simulink model "flightControlSystem"  (R2026b)
settings: Solver=ode3  StopTime=TFinal
PreLoadFcn:
  | InitVars;
undefined symbols (not defined in the file): control_power, feedforward_gains, integrator_limits, MC_PITCH_P, MC_PITCHRATE_D, MC_PITCHRATE_I, MC_PITCHRATE_MAX, MC_PITCHRATE_P, MC_ROLL_P, MC_ROLLRATE_D, MC_ROLLRATE_I, MC_ROLLRATE_MAX, MC_ROLLRATE_P, MC_YAW_P, MC_YAW_TQ_CUTOFF, MC_YAW_WEIGHT, MC_YAWRATE_D, MC_YAWRATE_I, MC_YAWRATE_MAX, MC_YAWRATE_P, MPC_ACC_DECOUPLE, MPC_LAND_ALT1, MPC_LAND_ALT2, MPC_LAND_ALT3, MPC_LAND_CRWL, MPC_LAND_SPEED, MPC_THR_HOVER, MPC_THR_MAX, MPC_THR_MIN, MPC_THR_XY_MARG, MPC_TILTMAX_AIR, MPC_VELD_LP, MPC_XY_P, MPC_XY_VEL_D_ACC, MPC_XY_VEL_I_ACC, MPC_XY_VEL_MAX, MPC_XY_VEL_P_ACC, MPC_Z_P, MPC_Z_VEL_D_ACC, MPC_Z_VEL_I_ACC, MPC_Z_VEL_MAX_DN, MPC_Z_VEL_MAX_UP, MPC_Z_VEL_P_ACC, SampleTime, timestamp
libraries: px4uORBlib x9, vrlib x8, aerolibutil x8, simulink x4, px4Utilslib x4, sharedutil x3, matrix_library x3, raspberrypiutilitieslib x2, px4Peripheralslib x2, sharedtransform x1, px4Sensorslib x1
(part 3 of 4)

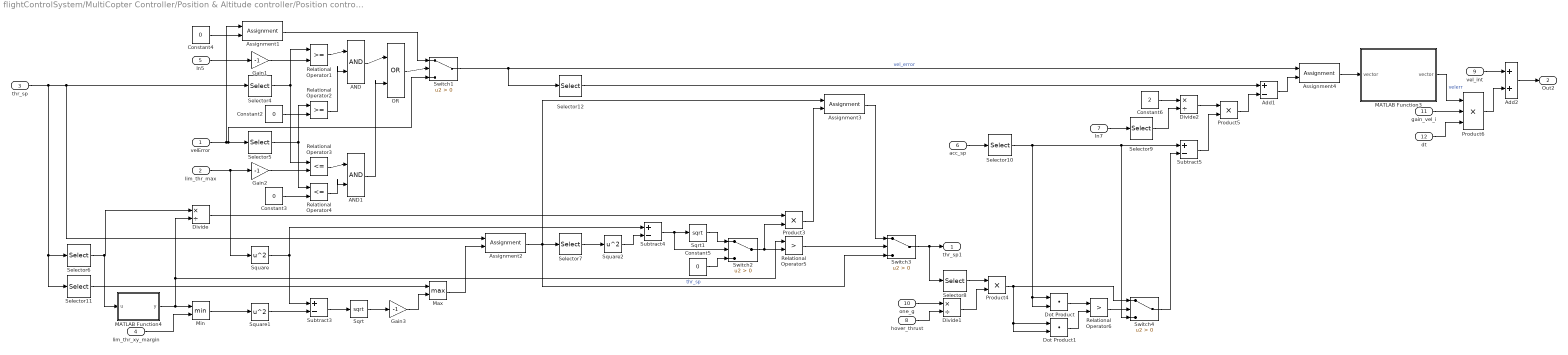
== system flightControlSystem/MultiCopter Controller/Position & Altitude controller/Position controller/Pos/thrust_allocation ==
  velError : Inport
  lim_thr_max : Inport  Port=2
  thr_sp : Inport  Port=3
  lim_thr_xy_margin : Inport  Port=4
  In5 : Inport  Port=5
  acc_sp : Inport  Port=6
  In7 : Inport  Port=7
  hover_thrust : Inport  Port=8
  vel_int : Inport  Port=9
  one_g : Inport  Port=10
  gain_vel_i : Inport  Port=11
  dt : Inport  Port=12
  AND : Logic  IconShape=distinctive  AllPortsSameDT=off  OutDataTypeStr=boolean
  AND1 : Logic  IconShape=distinctive  AllPortsSameDT=off  OutDataTypeStr=boolean
  Add1 : Sum  Inputs=+-
  Add2 : Sum
  Assignment1 : Assignment  DiagnosticForDimensions=Warning  IndexOptions=Index vector (dialog)  Indices=3  OutputSizes=1  RuntimeRangeChecks=off
  Assignment2 : Assignment  DiagnosticForDimensions=Warning  IndexOptions=Index vector (dialog)  Indices=3  OutputSizes=1  RuntimeRangeChecks=off
  Assignment3 : Assignment  DiagnosticForDimensions=Warning  IndexOptions=Index vector (dialog)  Indices=[1,2]  OutputSizes=1  RuntimeRangeChecks=off
  Assignment4 : Assignment  DiagnosticForDimensions=Warning  IndexOptions=Index vector (dialog)  Indices=[1 2]  OutputSizes=1  RuntimeRangeChecks=off
  Constant{2..5} (4 alike) : Constant  Value=0  SampleTime=-1
  Constant6 : Constant  Value=2  SampleTime=-1
  Divide : Product  Inputs=*/
  Divide1 : Product  Inputs=*/
  Divide2 : Product  Inputs=*/
  Dot Product : DotProduct  OutDataTypeStr=Inherit: Inherit via internal rule
  Dot Product1 : DotProduct  OutDataTypeStr=Inherit: Inherit via internal rule
  Gain1 : Gain  Gain=-1
  Gain2 : Gain  Gain=-1
  Gain3 : Gain  Gain=-1
  MATLAB Function3 : MATLAB Function  TreatAsAtomicUnit=on
  MATLAB Function4 : MATLAB Function  TreatAsAtomicUnit=on
  Max : MinMax  Function=max  Inputs=2
  Min : MinMax  Inputs=2
  OR : Logic  Operator=OR  IconShape=distinctive  AllPortsSameDT=off  OutDataTypeStr=boolean
  Product3 : Product
  Product4 : Product
  Product5 : Product
  Product6 : Product  Inputs=3
  Relational Operator1 : RelationalOperator  OutDataTypeStr=boolean  RndMeth=Simplest  InputSameDT=off
  Relational Operator2 : RelationalOperator  OutDataTypeStr=boolean  RndMeth=Simplest  InputSameDT=off
  Relational Operator3 : RelationalOperator  Operator=<=  OutDataTypeStr=boolean  RndMeth=Simplest  InputSameDT=off
  Relational Operator4 : RelationalOperator  Operator=<=  OutDataTypeStr=boolean  RndMeth=Simplest  InputSameDT=off
  Relational Operator5 : RelationalOperator  Operator=>  OutDataTypeStr=boolean  RndMeth=Simplest  InputSameDT=off
  Relational Operator6 : RelationalOperator  Operator=>  OutDataTypeStr=boolean  RndMeth=Simplest  InputSameDT=off
  Selector{6,8,10,12} (4 alike) : Selector  InputPortWidth=3  IndexOptions=Index vector (dialog)  Indices=[1 2]  OutputSizes=1  RuntimeRangeChecks=off
  Selector{4..5,7,11} (4 alike) : Selector  InputPortWidth=3  IndexOptions=Index vector (dialog)  Indices=3  OutputSizes=1  RuntimeRangeChecks=off
  Selector9 : Selector  InputPortWidth=3  IndexOptions=Index vector (dialog)  Indices=1  OutputSizes=1  RuntimeRangeChecks=off
  Sqrt : Sqrt
  Sqrt1 : Sqrt
  Square : Math  Operator=square
  Square1 : Math  Operator=square
  Square2 : Math  Operator=square
  Subtract3 : Sum  Inputs=+-
  Subtract4 : Sum  Inputs=+-
  Subtract5 : Sum  Inputs=+-
  Switch{1..4} (4 alike) : Switch  Criteria=u2 > Threshold  SaturateOnIntegerOverflow=off  InputSameDT=off
  thr_sp1 : Outport
  Out2 : Outport  Port=2
  wires:
  Assignment2/1 -> Assignment3/1, Switch3/3, Selector7/1  "thr_sp"
  thr_sp/1 -> Selector6/1, Selector11/1, Selector4/1, Assignment2/1
  Constant4/1 -> Assignment1/2
  MATLAB Function4/1(y) -> Relational Operator5/1, Divide/2, Min/1
  Divide2/1 -> Product5/1
  Min/1 -> Square1/1
  Selector6/1 -> Divide/1, MATLAB Function4/1(u)
  Constant6/1 -> Divide2/1
  Selector11/1 -> Max/1
  lim_thr_xy_margin/1 -> Min/2
  velError/1 -> Selector5/1, Switch1/3, Assignment1/1
  Selector12/1 -> Add1/1
  In5/1 -> Gain1/1
  lim_thr_max/1 -> Square/1, Gain2/1
  Switch4/1 -> Subtract5/2
  Divide/1 -> Product3/1
  Assignment1/1 -> Switch1/1
  In7/1 -> Selector9/1
  Gain1/1 -> Relational Operator1/2
  Selector4/1 -> Relational Operator3/1, Relational Operator1/1
  Constant2/1 -> Relational Operator2/2
  Selector5/1 -> Relational Operator4/1, Relational Operator2/1
  Gain2/1 -> Relational Operator3/2
  Relational Operator6/1 -> Switch4/2
  Switch2/1 -> Product3/2, Relational Operator5/2
  Constant3/1 -> Relational Operator4/2
  Square/1 -> Subtract4/1, Subtract3/1
  Square1/1 -> Subtract3/2
  Relational Operator1/1 -> AND/1
  Relational Operator2/1 -> AND/2
  Relational Operator3/1 -> AND1/1
  Relational Operator4/1 -> AND1/2
  Subtract3/1 -> Sqrt/1
  AND/1 -> OR/1
  AND1/1 -> OR/2
  Sqrt/1 -> Gain3/1
  Add2/1 -> Out2/1
  OR/1 -> Switch1/2
  Product5/1 -> Add1/2
  Gain3/1 -> Max/2
  Switch1/1 -> Assignment4/1, Selector12/1  "vel_error"
  Divide1/1 -> Product4/2
  Max/1 -> Assignment2/2
  Selector7/1 -> Square2/1
  Square2/1 -> Subtract4/2
  Subtract4/1 -> Switch2/2, Sqrt1/1
  Sqrt1/1 -> Switch2/1
  Constant5/1 -> Switch2/3
  Selector9/1 -> Divide2/2
  Product3/1 -> Assignment3/2
  acc_sp/1 -> Selector10/1
  Relational Operator5/1 -> Switch3/2
  Assignment3/1 -> Switch3/1
  Switch3/1 -> thr_sp1/1, Selector8/1
  Selector10/1 -> Dot Product/2, Dot Product/1, Switch4/3, Subtract5/1
  one_g/1 -> Divide1/1
  hover_thrust/1 -> Divide1/2
  Product4/1 -> Dot Product1/2, Dot Product1/1, Switch4/1
  Selector8/1 -> Product4/1
  Dot Product/1 -> Relational Operator6/1
  Dot Product1/1 -> Relational Operator6/2
  Subtract5/1 -> Product5/2
  Add1/1 -> Assignment4/2
  Assignment4/1 -> MATLAB Function3/1("vector ")
  MATLAB Function3/1(vector) -> Product6/1  "velerr"
  gain_vel_i/1 -> Product6/2
  dt/1 -> Product6/3
  vel_int/1 -> Add2/1
  Product6/1 -> Add2/2

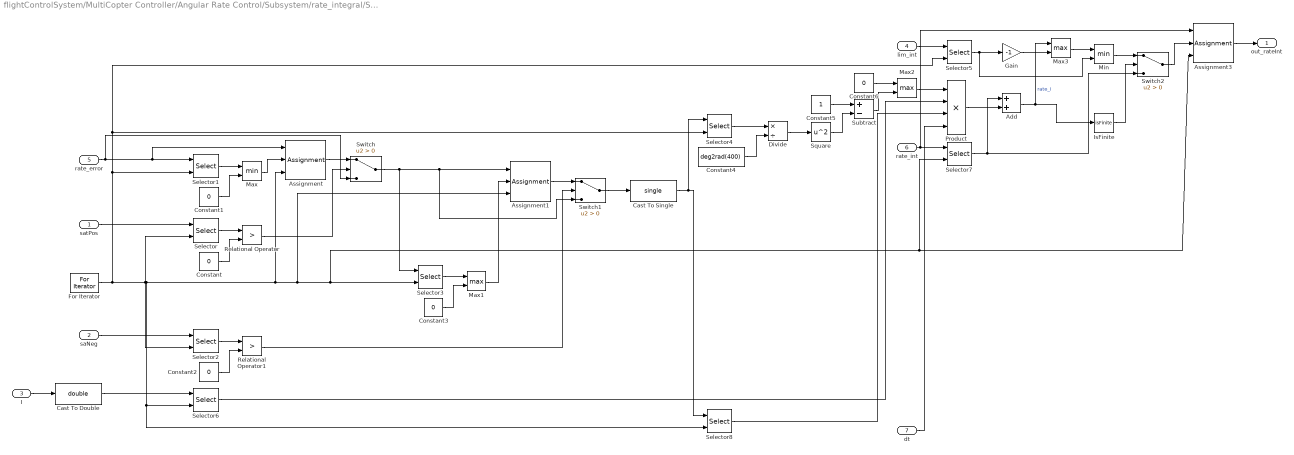
== system flightControlSystem/MultiCopter Controller/Angular Rate Control/Subsystem/rate_integral/Subsystem/Update_Integral ==
  satPos : Inport
  saNeg : Inport  Port=2
  I : Inport  Port=3
  lim_int : Inport  Port=4
  rate_error : Inport  Port=5
  rate_int : Inport  Port=6
  dt : Inport  Port=7
  Add : Sum
  Assignment : Assignment  DiagnosticForDimensions=Warning  IndexOptions=Index vector (port)  Indices=1  OutputSizes=1  RuntimeRangeChecks=off
  Assignment1 : Assignment  DiagnosticForDimensions=Warning  IndexOptions=Index vector (port)  Indices=1  OutputSizes=1  RuntimeRangeChecks=off
  Assignment3 : Assignment  DiagnosticForDimensions=Warning  IndexOptions=Index vector (port)  Indices=1  OutputSizes=1  RuntimeRangeChecks=off
  Cast To Double : DataTypeConversion  OutDataTypeStr=double  SaturateOnIntegerOverflow=off  RndMeth=Floor
  Cast To Single : DataTypeConversion  OutDataTypeStr=single  SaturateOnIntegerOverflow=off  RndMeth=Floor
  Constant{,1..3,6} (5 alike) : Constant  Value=0  SampleTime=-1
  Constant4 : Constant  Value=deg2rad(400)  SampleTime=-1
  Constant5 : Constant  SampleTime=-1
  Divide : Product  Inputs=*/
  For Iterator : ForIterator  IterationLimit=3
  Gain : Gain  Gain=-1
  IsFinite : RelationalOperator  Operator=isFinite  OutDataTypeStr=boolean  RndMeth=Simplest  InputSameDT=off
  Max : MinMax  Inputs=2
  Max1 : MinMax  Function=max  Inputs=2  OutDataTypeStr=double
  Max2 : MinMax  Function=max  Inputs=2
  Max3 : MinMax  Function=max  Inputs=2
  Min : MinMax  Inputs=2
  Product : Product  Inputs=4
  Relational Operator : RelationalOperator  Operator=>  OutDataTypeStr=boolean  RndMeth=Simplest  InputSameDT=off
  Relational Operator1 : RelationalOperator  Operator=>  OutDataTypeStr=boolean  RndMeth=Simplest  InputSameDT=off
  Selector{,1..8} (9 alike) : Selector  InputPortWidth=3  IndexOptions=Index vector (port)  Indices=[1 3]  OutputSizes=1  RuntimeRangeChecks=off
  Square : Math  Operator=square
  Subtract : Sum  Inputs=+-
  Switch : Switch  Criteria=u2 > Threshold  SaturateOnIntegerOverflow=off  InputSameDT=off
  Switch1 : Switch  Criteria=u2 > Threshold  SaturateOnIntegerOverflow=off  InputSameDT=off
  Switch2 : Switch  Criteria=u2 > Threshold  SaturateOnIntegerOverflow=off  InputSameDT=off
  out_rateInt : Outport
  wires:
  Switch/1 -> Switch1/3, Assignment1/1, Selector3/1
  I/1 -> Cast To Double/1
  rate_error/1 -> Assignment/1, Selector1/1, Switch/3
  Selector1/1 -> Max/1
  Selector7/1 -> Switch2/3, Add/1
  satPos/1 -> Selector/1
  Constant1/1 -> Max/2
  Subtract/1 -> Max2/2
  saNeg/1 -> Selector2/1
  For Iterator/1 -> Selector8/2, Selector6/2, Selector7/2, Assignment3/3, Selector3/2, Assignment1/3, Assignment/3, Selector2/2, Selector/2, Selector4/2, Selector5/2, Selector1/2
  Selector/1 -> Relational Operator/1
  Cast To Double/1 -> Selector6/1
  Constant/1 -> Relational Operator/2
  Selector2/1 -> Relational Operator1/1
  Constant2/1 -> Relational Operator1/2
  Selector6/1 -> Product/2
  Max/1 -> Assignment/2
  Relational Operator/1 -> Switch/2
  Relational Operator1/1 -> Switch1/2
  Assignment3/1 -> out_rateInt/1
  Assignment/1 -> Switch/1
  Selector3/1 -> Max1/1
  Constant3/1 -> Max1/2
  Max1/1 -> Assignment1/2
  Assignment1/1 -> Switch1/1
  Switch1/1 -> Cast To Single/1
  Cast To Single/1 -> Selector8/1, Selector4/1
  lim_int/1 -> Selector5/1
  Selector4/1 -> Divide/1
  Constant4/1 -> Divide/2
  IsFinite/1 -> Switch2/2
  Selector8/1 -> Product/3
  Divide/1 -> Square/1
  Constant5/1 -> Subtract/1
  Square/1 -> Subtract/2
  Constant6/1 -> Max2/1
  Max2/1 -> Product/1
  rate_int/1 -> Assignment3/1, Selector7/1
  dt/1 -> Product/4
  Selector5/1 -> Min/2, Gain/1
  Product/1 -> Add/2
  Gain/1 -> Max3/2
  Add/1 -> Max3/1, IsFinite/1  "rate_i"
  Max3/1 -> Min/1
  Min/1 -> Switch2/1
  Switch2/1 -> Assignment3/2

== system flightControlSystem/MultiCopter Controller/Position & Altitude controller/Position controller/Pos/Hover_Thrust/vel_int_constrain ==
  value : Inport
  max : Inport  Port=2
  min : Inport  Port=3
  Max : MinMax  Function=max  Inputs=2
  Min : MinMax  Inputs=2
  Out1 : Outport
  wires:
  value/1 -> Max/1
  min/1 -> Max/2
  Max/1 -> Min/1
  max/1 -> Min/2
  Min/1 -> Out1/1

== system flightControlSystem/MultiCopter Controller/Position & Altitude controller/Position controller/Pos/Position P control Loop/Subsystem ==
  "setpoint " : Inport
  addition : Inport  Port=2
  MATLAB Function : MATLAB Function  TreatAsAtomicUnit=on
  MATLAB Function1 : MATLAB Function  TreatAsAtomicUnit=on
  vector : Outport
  setpoint : Outport  Port=2
  wires:
  addition/1 -> MATLAB Function1/1("vector "), MATLAB Function/2(addition)
  MATLAB Function/1(setpoint) -> setpoint/1
  "setpoint "/1 -> MATLAB Function/1("setpoint ")
  MATLAB Function1/1(vector) -> vector/1

== system flightControlSystem/MultiCopter Controller/Position & Altitude controller/Position controller/Pos/Position P control Loop/constrain ==
  value : Inport
  min : Inport  Port=2
  max : Inport  Port=3
  Max : MinMax  Function=max  Inputs=2
  Min : MinMax  Inputs=2
  Out1 : Outport
  wires:
  value/1 -> Max/1
  min/1 -> Max/2
  Max/1 -> Min/1
  max/1 -> Min/2
  Min/1 -> Out1/1

== system flightControlSystem/MultiCopter Controller/Position & Altitude controller/Position controller/Pos/Position P control Loop/constrained_xy ==
  v0 : Inport
  v1 : Inport  Port=2
  max_val : Inport  Port=3
  Add : Sum
  Add1 : Sum
  Add2 : Sum
  Constant : Constant  Value=0.001  SampleTime=-1
  Constant1 : Constant  Value=0.001  SampleTime=-1
  Dot Product : DotProduct  OutDataTypeStr=Inherit: Inherit via internal rule
  Dot Product1 : DotProduct  OutDataTypeStr=Inherit: Inherit via internal rule
  Gain : Gain  Gain=-1
  MATLAB Function1 : MATLAB Function  TreatAsAtomicUnit=on
  MATLAB Function2 : MATLAB Function  TreatAsAtomicUnit=on
  MATLAB Function3 : MATLAB Function  TreatAsAtomicUnit=on
  MATLAB Function4 : MATLAB Function  TreatAsAtomicUnit=on
  Normalize Vector : vrlib/Utilities/Normalize Vector  maxzero=0
  Normalize Vector2 : vrlib/Utilities/Normalize Vector  maxzero=0
  Product1 : Product
  Product2 : Product
  Product3 : Product
  Relational Operator : RelationalOperator  Operator=<=  OutDataTypeStr=boolean  RndMeth=Simplest  InputSameDT=off
  Relational Operator1 : RelationalOperator  OutDataTypeStr=boolean  RndMeth=Simplest  InputSameDT=off
  Relational Operator2 : RelationalOperator  Operator=<  OutDataTypeStr=boolean  RndMeth=Simplest  InputSameDT=off
  Relational Operator3 : RelationalOperator  Operator=<  OutDataTypeStr=boolean  RndMeth=Simplest  InputSameDT=off
  Square : Math  Operator=square
  Square Root : Sqrt
  Square1 : Math  Operator=square
  Subtract : Sum  Inputs=+-
  Subtract1 : Sum  Inputs=+-
  Subtract2 : Sum  Inputs=+-
  Switch{,1..3} (4 alike) : Switch  Criteria=u2 > Threshold  SaturateOnIntegerOverflow=off  InputSameDT=off
  Out1 : Outport
  wires:
  Subtract/1 -> MATLAB Function4/1(u)
  v0/1 -> Add2/1, Dot Product1/1, Dot Product1/2, Dot Product/2, Add/1, MATLAB Function2/1(u), Subtract/2, Normalize Vector2/1, MATLAB Function1/1(u)
  v1/1 -> Add/2, Subtract/1, Normalize Vector/1
  MATLAB Function4/1(y) -> Relational Operator2/1
  max_val/1 -> Square/1, Product3/2, Product2/2, Relational Operator/2, Relational Operator1/2
  Normalize Vector/1 -> Product1/1, Product3/1, Dot Product/1
  Product3/1 -> Switch3/1
  MATLAB Function1/1(y) -> Relational Operator3/1
  Gain/1 -> Add1/1
  Normalize Vector2/1 -> Product2/1
  Constant1/1 -> Relational Operator3/2
  MATLAB Function2/1(y) -> Relational Operator1/1
  Relational Operator/1 -> Switch/2
  Add/1 -> Switch/1, MATLAB Function3/1(u)
  Square Root/1 -> Add1/2
  Dot Product/1 -> Gain/1, Square1/1
  Switch/1 -> Switch1/3
  Dot Product1/1 -> Subtract1/1
  Relational Operator2/1 -> Switch2/2
  Square/1 -> Subtract1/2
  Relational Operator3/1 -> Switch3/2
  Constant/1 -> Relational Operator2/2
  Relational Operator1/1 -> Switch1/2
  MATLAB Function3/1(y) -> Relational Operator/1
  Square1/1 -> Subtract2/1
  Subtract1/1 -> Subtract2/2
  Subtract2/1 -> Square Root/1
  Product2/1 -> Switch2/1, Switch1/1
  Add1/1 -> Product1/2
  Product1/1 -> Add2/2
  Add2/1 -> Switch/3
  Switch1/1 -> Switch2/3
  Switch3/1 -> Out1/1
  Switch2/1 -> Switch3/3

== system flightControlSystem/MultiCopter Controller/Position & Altitude controller/Position controller/Pos/acceleration_control/ACC_Decoupling ==
  In2 : Inport
  Constant : Constant  Value=9.81  OutDataTypeStr=double  SampleTime=-1
  Decouple_Switch : Switch  Threshold=1
  MPC_ACC_DECOUPLE : Constant  Value=MPC_ACC_DECOUPLE  SampleTime=-1
  Sum_coupled : Sum  Inputs=+-
  Out1 : Outport
  wires:
  MPC_ACC_DECOUPLE/1 -> Decouple_Switch/2
  Sum_coupled/1 -> Decouple_Switch/3
  In2/1 -> Sum_coupled/2
  Decouple_Switch/1 -> Out1/1
  Constant/1 -> Sum_coupled/1, Decouple_Switch/1

== system flightControlSystem/MultiCopter Controller/Position & Altitude controller/Position controller/Pos/acceleration_control/limitTilt ==
  body_unit : Inport
  world_unit : Inport  Port=2
  max_angle : Inport  Port=3
  Acos : Trigonometry  Operator=acos
  Add : Sum
  Assignment : Assignment  DiagnosticForDimensions=Warning  IndexOptions=Index vector (dialog)  Indices=1  OutputSizes=1  RuntimeRangeChecks=off
  Constant : Constant  Value=eps('single');  SampleTime=-1
  Constant1 : Constant  SampleTime=-1
  Cos : Trigonometry  Operator=cos
  Divide : Product  Inputs=*/
  Dot Product : DotProduct  OutDataTypeStr=Inherit: Inherit via internal rule
  Dot Product1 : DotProduct  OutDataTypeStr=Inherit: Inherit via internal rule
  MATLAB Function4 : MATLAB Function  TreatAsAtomicUnit=on
  Min : MinMax  Inputs=2
  Product : Product
  Product1 : Product
  Product2 : Product
  Relational Operator : RelationalOperator  Operator=<  OutDataTypeStr=boolean  RndMeth=Simplest  InputSameDT=off
  Sin : Trigonometry
  Subtract : Sum  Inputs=+-
  Switch : Switch  Criteria=u2 > Threshold  SaturateOnIntegerOverflow=off  InputSameDT=off
  Out1 : Outport
  wires:
  body_unit/1 -> Dot Product/1, Subtract/1
  world_unit/1 -> Product/2, Product1/2, Dot Product/2
  Dot Product/1 -> Acos/1, Product/1
  Acos/1 -> Min/1
  max_angle/1 -> Min/2
  Product/1 -> Subtract/2
  Constant/1 -> Relational Operator/2
  Subtract/1 -> Switch/3, Assignment/1, Dot Product1/1, Dot Product1/2
  Dot Product1/1 -> Relational Operator/1
  Relational Operator/1 -> Switch/2
  Constant1/1 -> Assignment/2
  Assignment/1 -> Switch/1
  Min/1 -> Sin/1, Cos/1
  Cos/1 -> Product1/1
  Sin/1 -> Product2/1
  MATLAB Function4/1(y) -> Divide/2
  Switch/1 -> MATLAB Function4/1(u), Divide/1
  Divide/1 -> Product2/2
  Product1/1 -> Add/1
  Product2/1 -> Add/2
  Add/1 -> Out1/1

== matlab function flightControlSystem/MultiCopter Controller/Angle_Control/AttitudeControl/vectorToQuaternion/norm ==
  data: u input; y output
function y = fcn(u)

y = norm(u);

== matlab function flightControlSystem/Actuator Commands/Simulation Actuator Commands/Mixer/MATLAB Function ==
  data: frameType input; rotor_cmd output size=[1 8]; thrust input; pitch input; roll input; yaw input
function rotor_cmd = MixerBlock(frameType, thrust, pitch, roll, yaw)
%#codegen
% Outputs a 1x8 vector for bus conversion

    rotor_cmd = zeros(1,8); % Always 8 motors

    % Select mixer matrix
    if frameType == "Quad+"
        mixer = [1,0,-1,1;
                 1,0,1,1;
                 1,1,0,-1;
                 1,-1,0,-1];
        N = 4;
    elseif frameType == "QuadX"
        mixer = [1,1,-1,1;
                 1,-1,1,1;
                 1,-1,-1,-1;
                 1,1,1,-1];
        N = 4;
    elseif frameType == "QuadH"
        mixer = [1,1,-1,1;
                 1,-1,1,1;
                 1,-1,-1,-1;
                 1,1,1,-1]; % Yaw    (from rotorDir)

        N = 4;
	elseif frameType == "Hexa+"
		s60 = sqrt(3)/2;
		c60 = 1/2;
		mixer = [
			1,  1,  0,  -1;           
			1, -1,  0,  1;           
			1, -0.5, -s60,  -1;            
			1,  0.5,  s60,  1;            
			1,  0.5, -s60,  1;            
			1, -0.5,  s60,  -1];           
		N = 6;
	elseif frameType == "HexaX"
		mixer = [
			1,  0,  1, -1;   
			1,  0, -1,  1;  
			1,  1, -1, -1;   
			1, -1,  1,  1;   
			1,  1,  1,  1;  
			1, -1, -1, -1    
			];
		N = 6;
    % elseif frameType == "OctoX"
    %     mixer = [1, 1, 0, 1;
    %              1, 0, -1, 1;
    %              1, -1, 0, 1;
    %              1, 0, 1, 1;
    %              1, 1, 0, -1;
    %              1, 0, -1, -1;
    %              1, -1, 0, -1;
    %              1, 0, 1, -1];
    %     N = 8;
    else
        mixer = zeros(4,4);
        N = 4;
    end

    ctrl = [thrust; pitch; roll; yaw];
    rotor = mixer * ctrl;
    rotor_cmd(1:N) = reshape(rotor,1,[]);
end

== matlab function flightControlSystem/MultiCopter Controller/Angle_Control/AttitudeControl/MATLAB Function7 ==
  data: q input; v output
function v = dcmZ(q)
    % Corresponding body z-axis to an attitude quaternion
    a = q(1);
    b = q(2);
    c = q(3);
    d = q(4);
    v = [2 * (a * c + b * d);
         2 * (c * d - a * b);
         a * a - b * b - c * c + d * d];
end

== matlab function flightControlSystem/MultiCopter Controller/Angle_Control/AttitudeControl/MATLAB Function ==
  data: q input; q_canonical output
function q_canonical = canonical(q)
    % Return canonical form of the quaternion
    % Iterate over quaternion elements to find the first non-negligible component
    % and use its sign to adjust the quaternion to its canonical form.

    epsilon = eps('single'); % Equivalent to FLT_EPSILON in C++
    
    for i = 1:4
        if abs(q(i)) > epsilon
            q_canonical = q * single(sign(q(i)));
            return;
        end
    end

    % If all components are negligible (unlikely for a valid quaternion),
    % return the original quaternion.
    q_canonical = single(q);
end

== matlab function flightControlSystem/MultiCopter Controller/Angle_Control/AttitudeControl/MATLAB Function2 ==
  data: q input; q_canonical output
function q_canonical = canonical(q)
    % Return canonical form of the quaternion
    % Iterate over quaternion elements to find the first non-negligible component
    % and use its sign to adjust the quaternion to its canonical form.

    epsilon = eps('single'); % Equivalent to FLT_EPSILON in C++
    
    for i = 1:4
        if abs(q(i)) > epsilon
            q_canonical = q * single(sign(q(i)));
            return;
        end
    end

    % If all components are negligible (unlikely for a valid quaternion),
    % return the original quaternion.
    q_canonical = single(q);
end

== matlab function flightControlSystem/MultiCopter Controller/Angle_Control/AttitudeControl/MATLAB Function3 ==
  data: q input; v output
function v = dcmZ(q)
    % Corresponding body z-axis to an attitude quaternion
    a = q(1);
    b = q(2);
    c = q(3);
    d = q(4);
    v = [2 * (a * c + b * d);
         2 * (c * d - a * b);
         a * a - b * b - c * c + d * d];
end

== matlab function flightControlSystem/MultiCopter Controller/Angle_Control/AttitudeControl/MATLAB Function4 ==
  data: q input; v output
function v = quatImag(q)
    % Imaginary part of quaternion
    v = q(2:4);
end

== matlab function flightControlSystem/MultiCopter Controller/Angular Rate Control/MATLAB Function ==
  data: vehicle_torque_setpoint input; dt input; control_power output
function control_power = updateActuatorControlsStatus(vehicle_torque_setpoint, dt)
	persistent control_energy energy_integration_time
	
	if isempty(control_energy)
		control_energy = zeros(1, 3);
		energy_integration_time = 0;
	end
	
	control_power = zeros(1, 3);
	
	% Update control energy
	for i = 1:3
		control_energy(i) = control_energy(i) + vehicle_torque_setpoint(i) * vehicle_torque_setpoint(i) * dt;
	end
	
	% Update energy integration time
	energy_integration_time = energy_integration_time + dt;
	
	% Check if integration time exceeds threshold
	if energy_integration_time > 500e-3
	
		for i = 1:3
			control_power(i) = control_energy(i) / energy_integration_time;
			control_energy(i) = 0;
		end

		% Reset integration time
		energy_integration_time = 0;
	end
end

== matlab function flightControlSystem/MultiCopter Controller/Angular Rate Control/Subsystem/YawTorqueLPF_v116 ==
  data: yaw_torque input; yaw_torque_filt output; dt input; MC_YAW_TQ_CUTOFF input
function yaw_torque_filt = YawTorqueLPF_v116(yaw_torque, dt, MC_YAW_TQ_CUTOFF)
%#codegen
% PX4 v1.16 yaw torque low-pass filter
% Insertion point: after rate controller PID, before actuator mixer
% Reference: MulticopterRateControl.cpp
%   torque_setpoint(2) = _output_lpf_yaw.update(torque_setpoint(2), dt)
%
% Uses same AlphaFilter formula as velocity LP:
%   b = 2*pi*fc*dt; a = b/(1+b); state = a*input + (1-a)*state

persistent yaw_lp_state initialized

if isempty(initialized)
    yaw_lp_state = 0;
    initialized = true;
end

% AlphaFilter::update(sample, dt)
b = 2*pi*MC_YAW_TQ_CUTOFF*dt;
a = b / (1 + b);
yaw_lp_state = a * yaw_torque + (1 - a) * yaw_lp_state;
yaw_torque_filt = yaw_lp_state;

== matlab function flightControlSystem/MultiCopter Controller/Position & Altitude controller/Position controller/Pos/Position P control Loop/Subsystem/MATLAB Function ==
  data: setpoint input; setpoint output; addition input
function setpoint = addIfNotNanVector3f(setpoint, addition)
    for i = 1:3
        setpoint(i) = addIfNotNan(setpoint(i), addition(i));
    end
end

function value = addIfNotNan(value, addition)
    value = single(value);
    if isfinite(value) && isfinite(addition)
        value = value + addition;
    elseif ~isfinite(value)
        value = single(addition);
    end
    % If addition is NaN or both are NaN, do nothing
end

== matlab function flightControlSystem/MultiCopter Controller/Angle_Control/MATLAB Function4 ==
  data: roll input; qd output; pitch input; yaw input
function qd = eulerToQuaternion(roll, pitch, yaw)
    % Convert roll, pitch, yaw (in radians) to a quaternion
    cr = cos(roll / 2);
    sr = sin(roll / 2);
    cp = cos(pitch / 2);
    sp = sin(pitch / 2);
    cy = cos(yaw / 2);
    sy = sin(yaw / 2);

    qd = [cr * cp * cy + sr * sp * sy, ...
          sr * cp * cy - cr * sp * sy, ...
          cr * sp * cy + sr * cp * sy, ...
          cr * cp * sy - sr * sp * cy];
	qd = qd / norm(qd);
end

== matlab function flightControlSystem/Actuator Commands/Actuator Commands/MATLAB Function ==
  data: y output
function y = fcn()

y =  zeros(1,8);

== matlab function flightControlSystem/get TargetGetAndSetpoint/Set target Position/Landing Logic/PX4 Landing Logic ==
  data: land_trigger input; pos_sp output; states input; MPC_LAND_SPEED_in input; MPC_LAND_CRWL_in input; MPC_LAND_ALT1_in input; MPC_LAND_ALT2_in input; MPC_LAND_ALT3_in input; MPC_Z_VEL_MAX_DN_in input; vel_sp output; acc_sp output
function [pos_sp, vel_sp, acc_sp] = PX4LandingLogic(land_trigger, states, MPC_LAND_SPEED_in, MPC_LAND_CRWL_in, MPC_LAND_ALT1_in, MPC_LAND_ALT2_in, MPC_LAND_ALT3_in, MPC_Z_VEL_MAX_DN_in)
%#codegen
% PX4 v1.16.2 style multi-phase landing logic
% states = [X, Y, Z, Yaw] from getcurrentState bus
% In this controller: POSITIVE Vz = DESCEND (more thrust reduction)

persistent X_lock Y_lock Yaw_lock triggered
if isempty(triggered)
    triggered = false;
    X_lock = 0;
    Y_lock = 0;
    Yaw_lock = 0;
end

% Capture X, Y, Yaw on rising edge of land_trigger
if land_trigger > 0 && ~triggered
    X_lock = states(1);
    Y_lock = states(2);
    Yaw_lock = states(4);
    triggered = true;
elseif land_trigger == 0
    triggered = false;
end

if land_trigger > 0
    % Compute altitude above ground (positive up)
    altitude = -states(3);  % NED: Z negative = above ground

    % Multi-phase descent speed (PX4 v1.16.2)
    if altitude > MPC_LAND_ALT1_in
        land_speed = MPC_Z_VEL_MAX_DN_in;
    elseif altitude > MPC_LAND_ALT2_in
        frac = (altitude - MPC_LAND_ALT2_in) / (MPC_LAND_ALT1_in - MPC_LAND_ALT2_in);
        land_speed = MPC_LAND_SPEED_in + frac * (MPC_Z_VEL_MAX_DN_in - MPC_LAND_SPEED_in);
    elseif altitude > MPC_LAND_ALT3_in
        land_speed = MPC_LAND_SPEED_in;
    else
        land_speed = MPC_LAND_CRWL_in;
    end

    % Position: lock X,Y; NaN for Z (velocity-controlled); lock Yaw
    pos_sp = [X_lock, Y_lock, nan, Yaw_lock];

    % Velocity: zero XY, positive Vz for descent
    vel_sp = [0, 0, land_speed];

    % Acceleration: zero (no feedforward)
    acc_sp = [0, 0, 0];
else
    pos_sp = [0, 0, 0, 0];
    vel_sp = [0, 0, 0];
    acc_sp = [0, 0, 0];
end
end

== matlab function flightControlSystem/MultiCopter Controller/Position & Altitude controller/Position controller/Pos/Position P control Loop/Subsystem/MATLAB Function1 ==
  data: vector input; vector output
function vector = setZeroIfNanVector3f(vector)
    vector = addIfNotNanVector3f(vector, [0; 0; 0]);
end

% Function to add if not NaN for a 3-element vector
function setpoint = addIfNotNanVector3f(setpoint, addition)
for i = 1:3
    setpoint(i) = addIfNotNan(setpoint(i), addition(i));
end
end

% Function to add if not NaN
function value = addIfNotNan(value, addition)
value = single(value);
if isfinite(value) && isfinite(addition)
    value = value + addition;
elseif ~isfinite(value)
    value = single(addition);
end
% If addition is NaN or both are NaN, do nothing
end

== matlab function flightControlSystem/MultiCopter Controller/Position & Altitude controller/Position controller/Pos/Position P control Loop/constrained_xy/MATLAB Function1 ==
  data: u input; y output
function y = fcn(u)

y = norm(u);

== matlab function flightControlSystem/MultiCopter Controller/Position & Altitude controller/Position controller/Pos/Position P control Loop/constrained_xy/MATLAB Function2 ==
  data: u input; y output
function y = fcn(u)

y = norm(u);

== matlab function flightControlSystem/MultiCopter Controller/Position & Altitude controller/Position controller/Pos/Position P control Loop/constrained_xy/MATLAB Function3 ==
  data: u input; y output
function y = fcn(u)

y = norm(u);

== matlab function flightControlSystem/MultiCopter Controller/Position & Altitude controller/Position controller/Pos/thrust_allocation/MATLAB Function3 ==
  data: vector input; vector output
function vector = setZeroIfNanVector3f(vector)
    vector = addIfNotNanVector3f(vector, [0; 0; 0]);
end

% Function to add if not NaN for a 3-element vector
function setpoint = addIfNotNanVector3f(setpoint, addition)
for i = 1:3
    setpoint(i) = addIfNotNan(setpoint(i), addition(i));
end
end

% Function to add if not NaN
function value = addIfNotNan(value, addition)
value = single(value);
if isfinite(value) && isfinite(addition)
    value = value + addition;
elseif ~isfinite(value)
    value = single(addition);
end
% If addition is NaN or both are NaN, do nothing
end

== matlab function flightControlSystem/get TargetGetAndSetpoint/Simulation Set target Position/Landing Logic/PX4 Landing Logic ==
  data: land_trigger input; pos_sp output; states input; MPC_LAND_SPEED_in input; MPC_LAND_CRWL_in input; MPC_LAND_ALT1_in input; MPC_LAND_ALT2_in input; MPC_LAND_ALT3_in input; MPC_Z_VEL_MAX_DN_in input; vel_sp output; acc_sp output
function [pos_sp, vel_sp, acc_sp] = PX4LandingLogic(land_trigger, states, MPC_LAND_SPEED_in, MPC_LAND_CRWL_in, MPC_LAND_ALT1_in, MPC_LAND_ALT2_in, MPC_LAND_ALT3_in, MPC_Z_VEL_MAX_DN_in)
%#codegen
% PX4 v1.16.2 style multi-phase landing logic
% states = [X, Y, Z, Yaw] from getcurrentState bus
% In this controller: POSITIVE Vz = DESCEND (more thrust reduction)

persistent X_lock Y_lock Yaw_lock triggered
if isempty(triggered)
    triggered = false;
    X_lock = 0;
    Y_lock = 0;
    Yaw_lock = 0;
end

% Capture X, Y, Yaw on rising edge of land_trigger
if land_trigger > 0 && ~triggered
    X_lock = states(1);
    Y_lock = states(2);
    Yaw_lock = states(4);
    triggered = true;
elseif land_trigger == 0
    triggered = false;
end

if land_trigger > 0
    % Compute altitude above ground (positive up)
    altitude = -states(3);  % NED: Z negative = above ground

    % Multi-phase descent speed (PX4 v1.16.2)
    if altitude > MPC_LAND_ALT1_in
        land_speed = MPC_Z_VEL_MAX_DN_in;
    elseif altitude > MPC_LAND_ALT2_in
        frac = (altitude - MPC_LAND_ALT2_in) / (MPC_LAND_ALT1_in - MPC_LAND_ALT2_in);
        land_speed = MPC_LAND_SPEED_in + frac * (MPC_Z_VEL_MAX_DN_in - MPC_LAND_SPEED_in);
    elseif altitude > MPC_LAND_ALT3_in
        land_speed = MPC_LAND_SPEED_in;
    else
        land_speed = MPC_LAND_CRWL_in;
    end

    % Position: lock X,Y; NaN for Z (velocity-controlled); lock Yaw
    pos_sp = [X_lock, Y_lock, nan, Yaw_lock];

    % Velocity: zero XY, positive Vz for descent
    vel_sp = [0, 0, land_speed];

    % Acceleration: zero (no feedforward)
    acc_sp = [0, 0, 0];
else
    pos_sp = [0, 0, 0, 0];
    vel_sp = [0, 0, 0];
    acc_sp = [0, 0, 0];
end
end

== matlab function flightControlSystem/Estimator/Estimator/MATLAB Function1 ==
  data: timestamp_sample input; dt output
function dt = calculateDeltaTime(timestamp_sample)

    persistent time_stamp_last_loop;

    % Initialize _time_stamp_last_loop if it's empty
    if isempty(time_stamp_last_loop)
        time_stamp_last_loop = hrt_absolute_time();
    end

    % Calculate dt with constraints
    dt = constrain(((timestamp_sample - time_stamp_last_loop) * 1e-6), 0.002, 0.04);

    % Update _time_stamp_last_loop for the next iteration
    time_stamp_last_loop = timestamp_sample;
end

function value = constrain(value, min_val, max_val)
    % Constrain the value between min_val and max_val
    value = max(min(value, max_val), min_val);
end

function abs_time_us = hrt_absolute_time()
    % Initialize a persistent variable to store the start time
    persistent start_time;
    
    % If this is the first call, set the start time using tic
    if isempty(start_time)
        start_time = tic;
    end
    
    % Get the elapsed time since the start in seconds
    elapsed_time_sec = toc(start_time);
    
    % Convert elapsed time to microseconds
    abs_time_us = elapsed_time_sec * 1e6;
end

== matlab function flightControlSystem/MultiCopter Controller/Position & Altitude controller/Position controller/Pos/Position P control Loop/constrained_xy/MATLAB Function4 ==
  data: u input; y output
function y = fcn(u)

y = norm(u);

== matlab function flightControlSystem/MultiCopter Controller/Position & Altitude controller/Position controller/Pos/IgnoreOpticalFlow_till_25cm/MATLAB Function ==
  data: vel_sp_z input; vel_sp_z_limited output; dt input
function vel_sp_z_limited = TakeoffRamp(vel_sp_z, dt)
%#codegen
%TakeoffRamp  PX4 v1.16 takeoff velocity ramp
%  This LIMITS the maximum upward velocity - it does NOT override the
%  position controller. The position controller still controls to target
%  altitude; this just prevents it from commanding too much climb rate
%  during the first few seconds (which causes thrust transient → drift).
%
%  vel_sp_z comes FROM the position P-controller (already computed from
%  altitude error). This block only clamps it, never makes it climb faster.

persistent state elapsed ramp_progress

COM_SPOOLUP_TIME = 1.0;   % Motor spool-up (seconds)
MPC_TKO_RAMP_T  = 3.0;    % Ramp duration (seconds)
MPC_TKO_SPEED   = 1.5;    % Max takeoff climb rate (m/s, positive up)
MPC_Z_VEL_P     = 4.0;    % Z velocity P-gain (your Constant8(3))

if isempty(state)
    state = uint8(0);       % 0=spoolup, 1=rampup, 2=flight
    elapsed = 0.0;
    ramp_progress = 0.0;
end

% Zero-thrust velocity: vel_sp that makes velocity PID output ≈ 0
ramp_vz_init = -9.81 / max(MPC_Z_VEL_P, 0.01);  % ≈ -2.45 m/s (NED)

switch state
    case uint8(0)
        % SPOOLUP: clamp to zero-thrust velocity (motors spinning up)
        % Position controller may want to climb, but we don't allow it yet
        vel_sp_z_limited = max(vel_sp_z, ramp_vz_init);
        elapsed = elapsed + dt;
        if elapsed >= COM_SPOOLUP_TIME
            state = uint8(1);
        end

    case uint8(1)
        % RAMPUP: gradually open the velocity limit
        if MPC_TKO_RAMP_T > 0
            ramp_progress = min(ramp_progress + dt / MPC_TKO_RAMP_T, 1.0);
        else
            ramp_progress = 1.0;
        end

        % Current velocity ceiling (interpolate from ramp_vz_init to -TKO_SPEED)
        vel_limit = ramp_vz_init + ramp_progress * (-MPC_TKO_SPEED - ramp_vz_init);

        % CLAMP: position controller's vel_sp cannot exceed this limit
        % In NED: more negative = faster climb. max() picks the slower (less negative).
        % If pos controller wants -0.5 m/s and limit is -1.0 → pass -0.5 (within limit)
        % If pos controller wants -3.0 m/s and limit is -1.0 → clamp to -1.0
        vel_sp_z_limited = max(vel_sp_z, vel_limit);

        if ramp_progress >= 1.0
            state = uint8(2);
        end

    case uint8(2)
        % FLIGHT: no limiting, position controller has full authority
        vel_sp_z_limited = vel_sp_z;

    otherwise
        vel_sp_z_limited = vel_sp_z;
end
end

== matlab function flightControlSystem/MultiCopter Controller/Position & Altitude controller/Position controller/Pos/Hover_Thrust/MATLAB Function5 ==
  data: az input; hover_thrust_estimate output; thrust input; dt input; vx input; vy input; vz input; mpc_hover_thrust input
function hover_thrust_estimate = hoverThrustEstimator(az, thrust, dt, vx, vy, vz, mpc_hover_thrust)
    % Constants
    CONSTANTS_ONE_G = single(9.81); % Gravity constant

    acc_z = az;
    % Persistent variables to maintain state across function calls
    persistent hover_thr hover_thr_min hover_thr_max gate_size state_var process_var acc_var acc_var_scale
    persistent innov innov_var innov_test_ratio residual_lpf signed_innov_test_ratio_lpf
    persistent noise_learning_time_constant lpf_time_constant valid param_updated

    mpc_thr_hover = mpc_hover_thrust;
    hte_thr_range = single(0.2);
    hte_vz_thr = single(2);
    hte_vxy_thr = single(10);
    hte_ht_noise = single(0.0036);
    hte_ht_err_init = single(0.1);
    hte_acc_gate = single(3);
    in_air = single(1);
    armed = single(1);

    if isempty(hover_thr)
        % Initialize parameters
        hover_thr = single(0.5);
        hover_thr_min = single(0.1);
        hover_thr_max = single(0.9);
        gate_size = single(3.0);
        state_var = single(0.01);
        process_var = single(12.5e-6);
        acc_var = single(5.0);
        acc_var_scale = single(1.0);
        innov = single(0.0);
        innov_var = single(0.0);
        innov_test_ratio = single(0.0);
        residual_lpf = single(0.0);
        signed_innov_test_ratio_lpf = single(0.0);
        noise_learning_time_constant = single(2.0);
        lpf_time_constant = single(1.0);
        valid = false;
    end

    % Update parameters if needed
    if isempty(param_updated)
        hover_thr_min = single(max(mpc_thr_hover - hte_thr_range, 0.0));
        hover_thr_max = single(min(mpc_thr_hover + hte_thr_range, 1.0));
        process_var = hte_ht_noise^2;
        state_var = hte_ht_err_init^2;
        gate_size = hte_acc_gate;
        param_updated = true;
    end

    % Check preconditions
    if armed && in_air && (dt > 0.001) && (dt < 1.0) && isfinite(az)
        % Predict step
        state_var = state_var + process_var * dt^2;

        % Calculate measurement noise coefficients
        meas_noise_coeff_z = max((abs(vz) - hte_vz_thr) + 1.0, 1.0);
        meas_noise_coeff_xy = max(norm_v([vx, vy]) - hte_vxy_thr + 1.0, 1.0);
        acc_var_scale = max(meas_noise_coeff_xy, meas_noise_coeff_z);

        % Measurement update
        H = -CONSTANTS_ONE_G * thrust / hover_thr^2;
        innov_var = max(H * state_var * H + acc_var * acc_var_scale, acc_var * acc_var_scale);
        predicted_acc_z = CONSTANTS_ONE_G * thrust / hover_thr - CONSTANTS_ONE_G;
        innov = acc_z - predicted_acc_z;
        K = state_var * H / innov_var;
        innov_test_ratio = innov^2 / (gate_size^2 * innov_var);

        % Update state if innovation test passes
        if innov_test_ratio < 1
            hover_thr = max(min(hover_thr + K * innov, hover_thr_max), hover_thr_min);
            state_var = max((1 - K * H) * state_var, 1e-10);
        elseif abs(signed_innov_test_ratio_lpf) > 0.2
            state_var = state_var + 1e3 * process_var * dt^2;
        end

        % Update low-pass filters
        alpha = dt / (lpf_time_constant + dt);
        residual = innov;
        residual_lpf = (1 - alpha) * residual_lpf + alpha * residual;
        signed_innov_test_ratio_lpf = (1 - alpha) * signed_innov_test_ratio_lpf + alpha * sign(innov) * innov_test_ratio;

        % Update measurement noise
        alpha = dt / (noise_learning_time_constant + dt);
        res_no_bias = residual - residual_lpf;
        acc_var = max((1 - alpha) * acc_var + alpha * (res_no_bias^2 + H * state_var * H), 1);

        % Update valid state
        if valid
            valid = valid && innov_test_ratio < 1;
        else
            valid = innov_test_ratio < 1 && state_var < 0.001;
        end
    end

    % Output the estimated hover thrust
    hover_thrust_estimate = hover_thr;
end

function v = norm_squared(v)
v = dot_v(v,v);
end

function v = length_v(v)
v = norm_v(v);
end

function v = norm_v(v)
v = sqrt(dot_v(v,v));
end

function v = unit_v(v)
v = v/norm_v(v);
end

function v = normalised_v(v)
v = unit_v(v);
end

function r = dot_v(a, b)
% a is a vector (1D array)
% b is a matrix
% The function computes the dot product of vector a with the first column of matrix b

% Ensure a is a column vector
a = a(:);

% Initialize the result
r = single(0);

% Get the number of elements in the vector
M = length(a);

% Compute the dot product with the first column of b
for i = 1:M
    r = r + a(i) * b(i);
end
end

== matlab function flightControlSystem/MultiCopter Controller/Position & Altitude controller/Position controller/Pos/thrust_allocation/MATLAB Function4 ==
  data: u input; y output
function y = fcn(u)

y = norm(u);

== matlab function flightControlSystem/get TargetGetAndSetpoint/Set target Position/RC Failsafe Signal/MATLAB Function ==
  data: status input; out output; ch8 input; RSSI input
function out = rcLatch(status, ch8, RSSI)
%#codegen
% Inputs:
%   status - scalar (e.g., uint8 or double)
%   ch8    - scalar (e.g., uint16 or double)
%   RSSI   - scalar (e.g., uint8 or double)
% Output:
%   out    - scalar (0 or 1)

persistent prevOut
if isempty(prevOut)
    prevOut = 0;
end

if status == 0 && RSSI ~= 0
    if ch8 > 1600
        prevOut = 1;
    elseif ch8 < 1600
        prevOut = 0;
    end
end

out = prevOut;
end

== matlab function flightControlSystem/MultiCopter Controller/Position & Altitude controller/Position controller/Pos/Velocity_Control/MATLAB Function2 ==
  data: setpoint input; setpoint output; addition input
% Function to add if not NaN for a 3-element vector
function setpoint = addIfNotNanVector3f(setpoint, addition)
    for i = 1:3
        setpoint(i) = addIfNotNan(setpoint(i), addition(i));
    end
end

% Function to add if not NaN
function value = addIfNotNan(value, addition)
	value = single(value);
    if isfinite(value) && isfinite(addition)
        value = value + addition;
    elseif ~isfinite(value)
        value = single(addition);
    end
    % If addition is NaN or both are NaN, do nothing
end

== matlab function flightControlSystem/MultiCopter Controller/Position & Altitude controller/Position controller/Pos/acceleration_control/limitTilt/MATLAB Function4 ==
  data: u input; y output
function y = fcn(u)

y = norm(u);

== matlab function flightControlSystem/Estimator/Estimator/MATLAB Function2 ==
  data: timestamp_sample input; dt output
function dt = calculateDeltaTime(timestamp_sample)

    persistent time_stamp_last_loop;

    % Initialize _time_stamp_last_loop if it's empty
    if isempty(time_stamp_last_loop)
        time_stamp_last_loop = hrt_absolute_time();
    end

    % Calculate dt with constraints
    dt = constrain(((timestamp_sample - time_stamp_last_loop) * 1e-6), 0.002, 0.02);

    % Update _time_stamp_last_loop for the next iteration
    time_stamp_last_loop = timestamp_sample;
end

function value = constrain(value, min_val, max_val)
    % Constrain the value between min_val and max_val
    value = max(min(value, max_val), min_val);
end

function abs_time_us = hrt_absolute_time()
    % Initialize a persistent variable to store the start time
    persistent start_time;
    
    % If this is the first call, set the start time using tic
    if isempty(start_time)
        start_time = tic;
    end
    
    % Get the elapsed time since the start in seconds
    elapsed_time_sec = toc(start_time);
    
    % Convert elapsed time to microseconds
    abs_time_us = elapsed_time_sec * 1e6;
end

== matlab function flightControlSystem/MultiCopter Controller/Position & Altitude controller/Position controller/thrustToAttitude/MATLAB Function ==
  data: body_x input; y output; body_y input; body_z input
function y = fcn(body_x, body_y, body_z)

y = rotm2eul([body_x, body_y, body_z],'ZYX');

== matlab function flightControlSystem/MultiCopter Controller/Position & Altitude controller/Position controller/MATLAB Function1 ==
  data: dt input; tilt_limit_deg input; lim_tilt output
function lim_tilt = updateSlewRateYaw(dt, tilt_limit_deg)
    % Define persistent variables to hold state across function calls
    persistent value slewrate
    
    % Initialize persistent variables on the first call
    if isempty(value)
        value = 0; % Initial value
    end
    if isempty(slewrate)
        slewrate = 0.2; % Slew rate
    end
    
    % Convert tilt limit from degrees to radians
    tilt_limit_rad = deg2rad(tilt_limit_deg);
    new_value = tilt_limit_rad;
    % Update slewrate with yaw wrapping [-pi, pi]
    d_wrapped = wrap_pi(new_value - value);
    updated_value = wrap_pi(updateSlewRate(value + d_wrapped, dt));
    
    % Update the persistent value
    value = updated_value;
    
    % Assign the updated value to lim_tilt
    lim_tilt = value;
end

function updated_value = updateSlewRate(new_value, dt)
    % Define persistent variables for the SlewRate function
    persistent value slewrate
    
    % Initialize persistent variables on the first call
    if isempty(value)
        value = 0; % Initial value
    end
    if isempty(slewrate)
        slewrate = 0.2; % Slew rate
    end
    
    % Limit the rate of change of the value
    dvalue_desired = new_value - value;
    dvalue_max = slewrate * dt;
    dvalue = constrain(dvalue_desired, -dvalue_max, dvalue_max);
    
    % Update the persistent value
    value = value + dvalue;
    updated_value = value;
end

function result = constrain(value, min_val, max_val)
    % Constrain value between min_val and max_val
    result = min(max(value, min_val), max_val);
end

function wrapped_angle = wrap_pi(angle)
    % Wrap the angle to the range [-π, π)

    % Define the low and high bounds
    low = -pi;
    high = pi;

    % Calculate the range
    range = high - low;

    % Check if the angle is already within the desired range
    if low <= angle && angle < high
        wrapped_angle = angle;
        return;
    end

    % Calculate the number of wraps and adjust the angle
    num_wraps = floor((angle - low) / range);
    wrapped_angle = angle - range * num_wraps;
end

== matlab function flightControlSystem/MultiCopter Controller/Position & Altitude controller/Position controller/thrustToAttitude/MATLAB Function4 ==
  data: u input; y output
function y = fcn(u)

y = norm(u);

== matlab function flightControlSystem/Estimator/Estimator/MATLAB Function4 ==
  data: timestamp_sample input; dt output
function dt = calculateDeltaTime(timestamp_sample)

    persistent time_stamp_last_loop;

    % Initialize _time_stamp_last_loop if it's empty
    if isempty(time_stamp_last_loop)
        time_stamp_last_loop = hrt_absolute_time();
    end

    % Calculate dt with constraints
    dt = constrain(((timestamp_sample - time_stamp_last_loop) * 1e-6), 0.002, 0.04);

    % Update _time_stamp_last_loop for the next iteration
    time_stamp_last_loop = timestamp_sample;
end

function value = constrain(value, min_val, max_val)
    % Constrain the value between min_val and max_val
    value = max(min(value, max_val), min_val);
end

function abs_time_us = hrt_absolute_time()
    % Initialize a persistent variable to store the start time
    persistent start_time;
    
    % If this is the first call, set the start time using tic
    if isempty(start_time)
        start_time = tic;
    end
    
    % Get the elapsed time since the start in seconds
    elapsed_time_sec = toc(start_time);
    
    % Convert elapsed time to microseconds
    abs_time_us = elapsed_time_sec * 1e6;
end

== matlab function flightControlSystem/Estimator/Simulation Estimator/MATLAB Function ==
  settings: updateMethod=DISCRETE
  data: u input; dt output
function dt = compute_dt(u)
%#codegen
persistent t_prev
if isempty(t_prev)
    t_prev = 0;
end

t_now = u;
dt = t_now - t_prev;
t_prev = t_now;

== matlab function flightControlSystem/MultiCopter Controller/Angle_Control/AttitudeControl/MATLAB Function1 ==
  data: q input; v output
function v = dcmZ(q)
    % Corresponding body z-axis to an attitude quaternion
    a = q(1);
    b = q(2);
    c = q(3);
    d = q(4);
    v = [2 * (a * c + b * d);
         2 * (c * d - a * b);
         a * a - b * b - c * c + d * d];
end

== matlab function flightControlSystem/Estimator/Simulation Estimator/MATLAB Function1 ==
  data: control_setpoint input; unallocated_torque output; torque_setpoint_achieved output
function [unallocated_torque, torque_setpoint_achieved] = ctrl_allocator(control_setpoint)

control_allocation_scale =([1,1,1]);
effectiveness = ([1,1,1]);
actuator_sp = ([0,0,0]);
actuator_trim = ([0,0,0]);
allocated_control = (effectiveness .* (actuator_sp - actuator_trim)) .* control_allocation_scale;
unallocated_control = control_setpoint - allocated_control;

unallocated_torque = unallocated_control(1:3);
torque_setpoint_achieved = norm(unallocated_torque)^2 < 1e-6;
end

== matlab function flightControlSystem/MultiCopter Controller/Angle_Control/AttitudeControl/vectorToQuaternion/MATLAB Function ==
  data: src input; q output; dst input
function q = quatFromVectors(src, dst)
    % Quaternion from two vectors using single precision
    eps = single(1e-5);
    
    src = single(src(:)); % Ensure column vector and single precision
    dst = single(dst(:)); % Ensure column vector and single precision

    cr = cross(src, dst);
    dt = dot(src, dst);

	if norm(cr) < eps && dt < 0
		% Handle 180 degree rotation
		cr = abs(src);
		if cr(1) < cr(2)
			if cr(1) < cr(3)
				cr = single([1; 0; 0]);
			else
				cr = single([0; 0; 1]);
			end
		else
			if cr(2) < cr(3)
				cr = single([0; 1; 0]);
			else
				cr = single([0; 0; 1]);
			end
		end
		q0 = single(0);
		cr = cross(src, cr);
	else
		% Normal case, do half-way quaternion solution
		q0 = dt + sqrt(dot(src,src) * dot(dst,dst));
	end

    q = single([q0; cr(1); cr(2); cr(3)]);
end
